simulink model "MrasObserverTest"  (R2026b)
settings: Solver=FixedStepDiscrete  StopTime=mrasTestCfg.Duration  FixedStep=mrasCfg.Ts
PostLoadFcn:
  | addpath(fullfile(fileparts(get_param(bdroot,'FileName')),'..','build_process'));initialize_mras_test(bdroot);
model workspace (MAT data in the model file):
  fixtureTruth.time = [0 5e-05 0.0001 0.00015 0.0002 0.00025 0.0003 0.00035 0.0004 0.00045 0.0005 0.00055 ... (10001 elements, 10001x1)]
  fixtureTruth.theta = [0.7 0.73 0.76 0.79 0.82 0.85 0.88 0.91 0.94 0.97 1 1.03 ... (10001 elements, 10001x1)]
  fixtureTruth.omega = [600 600 600 600 600 600 600 600 600 600 600 600 ... (10001 elements, 10001x1)]
  fixtureTruth.current = [-1.28843537448 -1.33373927001 -1.37784289022 -1.42070654484 -1.46229165945 -1.50256081028 -1.5414777578 -1.57900747938 -1.61511620081 -1.64977142668 -1.68294196962 -1.71459797838 ... (20002 elements, 10001x2)]
  fixtureTruth.voltage = [-15.090599744 -15.5653412529 -16.0260750053 -16.472386372 -16.9038737027 -17.3201486881 -17.7208367088 -18.1055771726 -18.4740238389 -18.8258451308 -19.1607244328 -19.4783603761 ... (20002 elements, 10001x2)]
  fixtureTruth.id = [0 0 0 0 0 0 0 0 0 0 0 0 ... (10001 elements, 10001x1)]
  fixtureTruth.iq = [2 2 2 2 2 2 2 2 2 2 2 2 ... (10001 elements, 10001x1)]
  fixtureTruth.motor.Ts = 5e-05
  fixtureTruth.motor.Rs = 0.5
  fixtureTruth.motor.L = 0.001
  fixtureTruth.motor.Flux = 0.035
  fixtureTruth.motor.PolePairs = 4
  fixtureTruth.motor.BandwidthHz = 30
  fixtureTruth.motor.Damping = 0.7
  fixtureTruth.motor.Kaw = 20
  fixtureTruth.motor.ResidualCutoffHz = 500
  fixtureTruth.motor.InitialAngle = 0
  fixtureTruth.motor.InitialOmega = 300
  fixtureTruth.motor.MinBootstrapOmega = 20
  fixtureTruth.motor.MaxOmega = 2000
  fixtureTruth.motor.MinOmega = 30
  fixtureTruth.motor.MinEmf = 1
  fixtureTruth.motor.MaxNormalizedD = 0.12
  fixtureTruth.motor.MaxNormalizedQ = 0.3
  fixtureTruth.motor.QualificationTime = 0.02
  fixtureTruth.motor.Kp = 263.893782902
  fixtureTruth.motor.Ki = 35530.5758439
  fixtureTruth.motor.ResidualAlpha = 0.135755248164
  fixtureTruth.motor.QualificationSamples = 400
  fixtureTruth.motor.Settings = [5e-05; 0.5; 0.001; 0.035; 263.893782902; 35530.5758439; 20; 0.135755248164; 0; 300; 20; 2000; 30; 1; 0.12; 0.3; 400]
  fixtureTruth.direction_prior = [1 1 1 1 1 1 1 1 1 1 1 1 ... (10001 elements, 10001x1)]
  mrasCfg.Ts = 5e-05
  mrasCfg.Rs = 0.5
  mrasCfg.L = 0.001
  mrasCfg.Flux = 0.035
  mrasCfg.PolePairs = 4
  mrasCfg.BandwidthHz = 30
  mrasCfg.Damping = 0.7
  mrasCfg.Kaw = 20
  mrasCfg.ResidualCutoffHz = 500
  mrasCfg.InitialAngle = 0
  mrasCfg.InitialOmega = 300
  mrasCfg.MinBootstrapOmega = 20
  mrasCfg.MaxOmega = 2000
  mrasCfg.MinOmega = 30
  mrasCfg.MinEmf = 1
  mrasCfg.MaxNormalizedD = 0.12
  mrasCfg.MaxNormalizedQ = 0.3
  mrasCfg.QualificationTime = 0.02
  mrasCfg.Kp = 263.893782902
  mrasCfg.Ki = 35530.5758439
  mrasCfg.ResidualAlpha = 0.135755248164
  mrasCfg.QualificationSamples = 400
  mrasCfg.Settings = [5e-05; 0.5; 0.001; 0.035; 263.893782902; 35530.5758439; 20; 0.135755248164; 0; 300; 20; 2000; 30; 1; 0.12; 0.3; 400]
  mrasTestCfg.Duration = 0.5
  mrasTestCfg.InitialAngle = 0.7
  mrasTestCfg.ElectricalSpeed = 600
  mrasTestCfg.Id = 0
  mrasTestCfg.Iq = 2
  mrasTestCfg.Direction = 1
  mrasTestCfg.Enable = 1
  mrasTestCfg.Reset = 0
  mrasTestCfg.NoiseRms = 0
  mrasTestCfg.NoiseSeed = 42
  mrasTestCfg.CheckStart = 0.35
  mrasTestCfg.CurrentDelay = 0
  mrasTestCfg.AngleRmsLimit = 0.08
  mrasTestCfg.SpeedRmsLimit = 8
  mrasTestCfg.ValidFractionMinimum = 0.95
  testStim.time = [0 5e-05 0.0001 0.00015 0.0002 0.00025 0.0003 0.00035 0.0004 0.00045 0.0005 0.00055 ... (10001 elements, 10001x1)]
  testStim.signals.values = [-15.090599744 -15.5653412529 -16.0260750053 -16.472386372 -16.9038737027 -17.3201486881 -17.7208367088 -18.1055771726 -18.4740238389 -18.8258451308 -19.1607244328 -19.4783603761 ... (90009 elements, 10001x9)]
  testStim.signals.dimensions = 9
libraries: MrasObserver x1
settings Model: Creator=24322  LastModifiedBy=24322

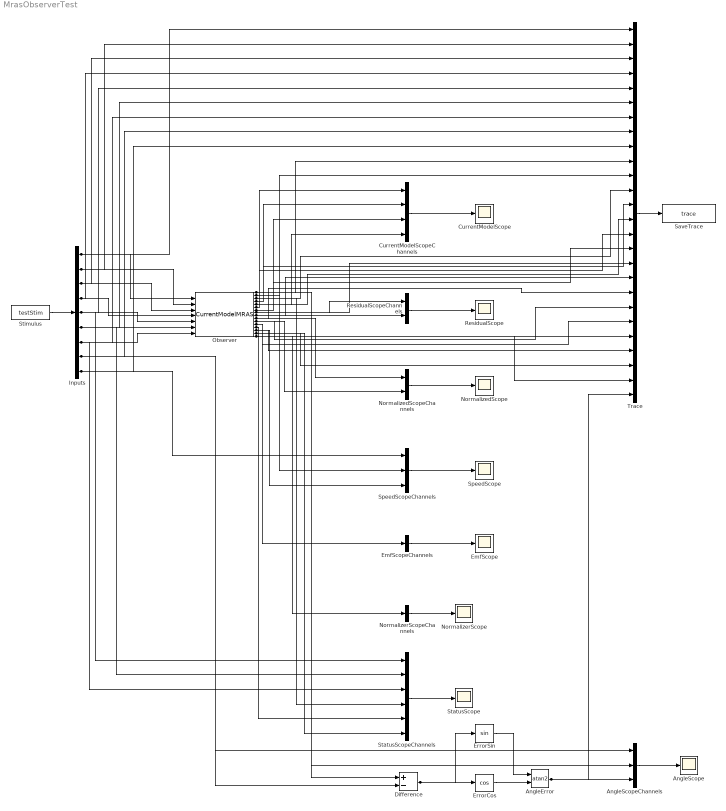
== system MrasObserverTest ==
  AngleError : Trigonometry  Operator=atan2
  AngleScope : Scope
  AngleScopeChannels : Mux  Inputs=3
  CurrentModelScope : Scope
  CurrentModelScopeChannels : Mux
  Difference : Sum  Inputs=+-
  EmfScope : Scope
  EmfScopeChannels : Mux  Inputs=1
  ErrorCos : Trigonometry  Operator=cos
  ErrorSin : Trigonometry
  Inputs : Demux  Outputs=9
  NormalizedScope : Scope
  NormalizedScopeChannels : Mux  Inputs=2
  NormalizerScope : Scope
  NormalizerScopeChannels : Mux  Inputs=1
  Observer : MrasObserver/CurrentModelMRAS  cfg=mrasCfg
  ResidualScope : Scope
  ResidualScopeChannels : Mux  Inputs=2
  SaveTrace : ToWorkspace  VariableName=trace  SaveFormat=Structure With Time  SampleTime=mrasCfg.Ts
  SpeedScope : Scope
  SpeedScopeChannels : Mux  Inputs=3
  StatusScope : Scope
  StatusScopeChannels : Mux  Inputs=6
  Stimulus : FromWorkspace  VariableName=testStim  SampleTime=mrasCfg.Ts  Interpolate=off  OutputAfterFinalValue=Holding final value
  Trace : Mux  Inputs=26
  wires:
  StatusScopeChannels/1 -> StatusScope/1
  NormalizerScopeChannels/1 -> NormalizerScope/1
  EmfScopeChannels/1 -> EmfScope/1
  NormalizedScopeChannels/1 -> NormalizedScope/1
  ResidualScopeChannels/1 -> ResidualScope/1
  CurrentModelScopeChannels/1 -> CurrentModelScope/1
  SpeedScopeChannels/1 -> SpeedScope/1
  AngleScopeChannels/1 -> AngleScope/1
  Observer/16 -> Trace/25, NormalizerScopeChannels/1
  Observer/15 -> Trace/24, StatusScopeChannels/6
  Observer/14 -> Trace/23, SpeedScopeChannels/3
  Observer/13 -> Trace/22, StatusScopeChannels/5
  Observer/12 -> Trace/21, EmfScopeChannels/1
  Observer/11 -> Trace/20, NormalizedScopeChannels/2
  Observer/10 -> Trace/19, NormalizedScopeChannels/1
  Observer/9 -> Trace/18, ResidualScopeChannels/2
  Observer/8 -> Trace/17, ResidualScopeChannels/1
  Observer/7 -> Trace/16, CurrentModelScopeChannels/3
  Observer/6 -> Trace/15, CurrentModelScopeChannels/1
  Observer/5 -> Trace/14, CurrentModelScopeChannels/4
  Observer/4 -> Trace/13, CurrentModelScopeChannels/2
  Observer/3 -> Trace/12, StatusScopeChannels/4
  Observer/2 -> Trace/11, SpeedScopeChannels/2
  Inputs/9 -> Trace/9, SpeedScopeChannels/1
  Inputs/7 -> Observer/7, Trace/7, StatusScopeChannels/3
  Inputs/6 -> Observer/6, Trace/6, StatusScopeChannels/2
  Inputs/5 -> StatusScopeChannels/1, Observer/5, Trace/5
  Inputs/4 -> Observer/4, Trace/4
  Inputs/3 -> Observer/3, Trace/3
  Inputs/2 -> Observer/2, Trace/2
  Inputs/1 -> Observer/1, Trace/1
  Trace/1 -> SaveTrace/1
  AngleError/1 -> Trace/26, AngleScopeChannels/3
  ErrorCos/1 -> AngleError/2
  ErrorSin/1 -> AngleError/1
  Difference/1 -> ErrorSin/1, ErrorCos/1
  Inputs/8 -> Trace/8, Difference/2, AngleScopeChannels/1
  Observer/1 -> Difference/1, Trace/10, AngleScopeChannels/2
  Stimulus/1 -> Inputs/1
